simulink model "L2_scheme"  (R2025a)
settings: Solver=VariableStepAuto  StartTime=0.0  StopTime=10.0  RelTol=1e-3

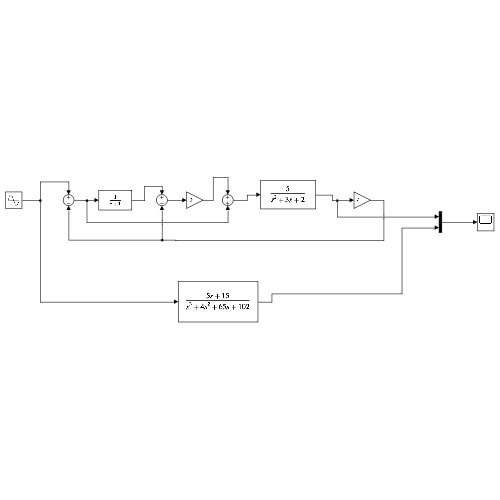
[thumbnail: Simulink's stored preview of the top-level diagram]
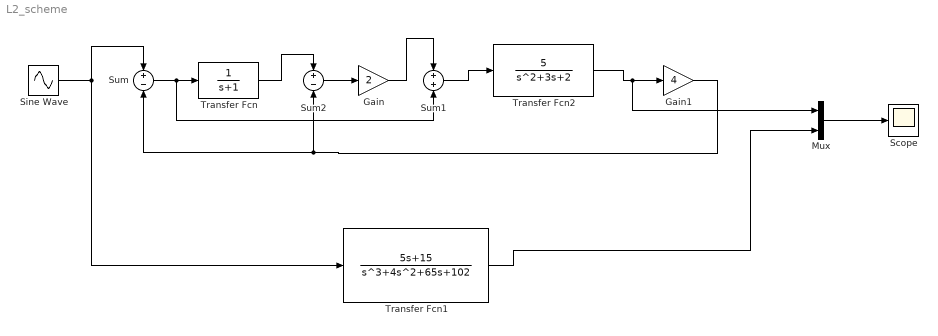
== system L2_scheme ==
  Gain : Gain  Gain=2
  Gain1 : Gain  Gain=4
  Mux : Mux  Inputs=2
  Scope : Scope
      settings: ActiveDisplayYMinimum=-0.15169992213404651  ActiveDisplayYMaximum=0.15786189793312649
  Sine Wave : Sin  Frequency=2  SampleTime=0
  Sum : Sum  Inputs=+-
  Sum1 : Sum
  Sum2 : Sum  Inputs=+-
  Transfer Fcn : TransferFcn  Denominator=[1 1]
  Transfer Fcn1 : TransferFcn  Numerator=[5 15]  Denominator=[1 4 65 102]
  Transfer Fcn2 : TransferFcn  Numerator=[5]  Denominator=[1 3 2]
  wires:
  Sine Wave/1 -> Sum/1, Transfer Fcn1/1
  Sum/1 -> Transfer Fcn/1, Sum1/2
  Transfer Fcn/1 -> Sum2/1
  Sum2/1 -> Gain/1
  Gain/1 -> Sum1/1
  Sum1/1 -> Transfer Fcn2/1
  Transfer Fcn2/1 -> Mux/1, Gain1/1
  Gain1/1 -> Sum/2, Sum2/2
  Transfer Fcn1/1 -> Mux/2
  Mux/1 -> Scope/1
